simulink model "sm_car"  (R2025a)
settings: Solver=ode23t  StartTime=0.0  StopTime=400  MaxStep=0.4  RelTol=1e-3  AbsTol=1e-3  EnableMultiTasking=on
PreLoadFcn:
  | % Due to usability issue in Repeating Sequence block
  | warning('off','Simulink:Masking:Invalid');
  | 
  | % Eliminate unnecessary warnings in inactive variants
  | % Warnings generated only if you click through inactive variant
  | warning('off','MATLAB:nonExistentField');
  | warning('off','Simulink:Parameters:BlkParamUndefined');
PostLoadFcn:
  | set_param([bdroot '/Vehicle'],'popup_trailer','Off')
  | warning('off','sm:sli:setup:compile:LocalSolverNotSupported')
  | %sm_car_config_maneuver(bdroot,'WOT Braking');
  | sm_car_config_vehicle(bdroot,'false');
  | sm_car_config_logging(bdroot);
InitFcn:
  | sm_car_config_camera;
  | Vehicle = sm_car_vehcfg_checkConfig(Vehicle);
  | sm_car_check_tire_model(bdroot);
StartFcn:
  | tic;
StopFcn:
  | Elapsed_Sim_Time = toc;
  | % disp(['Elapsed Sim Time = ' num2str(Elapsed_Sim_Time)]);
undefined symbols (not defined in the file): Axle1D, AxleIn, Camera, Control, Driver, Free, Init, Maneuver, Pedal, RaceFix, RaceSpin, Scene, ShaftL1, ShaftL2, ShaftR1, ShaftR2, Soft, Stiff, Visual, X, xy_data_car_side, Y, Z
libraries: sm_lib x1546, nesl_utility x528, fl_lib x480, SimscapeFluids_lib x61, sdl_lib x49, simulink x29, ee_lib x7, simulink_extras x6, Linkage_Systems x4, Tire_1x2x x4, AntiRollBar_Systems x2, Linkage_Decoupled x2
(part 7 of 79)

== system sm_car/Driver/Closed Loop/Maneuver/PoseTarget Visual ==
  note: Allow yaw angle to wrap for
      | clockwise and counterclockwise laps.
  ref_z : Inport
  ref_y : Inport  Port=2
  ref_x : Inport  Port=3
  Lap Count : Inport  Port=4
  ref_ayaw : Inport  Port=5
  CW or CCW : Constant  Value=sign(Maneuver.Trajectory.aYaw.Value(end)-Maneuver.Trajectory.aYaw.Value(1))
  Gain : Gain  Gain=2*pi
  MechanismConfiguration : sm_lib/Utilities/Mechanism Configuration  UniformGravity=None  GravityVector=[0 0 -9.80665]  GravityVectorUnits=m/s^2  LinearizationDelta=0.001  JointModeTransitionNonlinearIterations=2
  Pace Car : Subsystem  mask(Car Body Geometry){whl_cutout_rad=0.5, whl_base=abs(Vehicle.Chassis.Body.sAxle1.Value(1)-Vehicle.Chassis.Body.sAxle2.Value(1)), thk_top=0.05, thk_side=0.05, car_track=Vehicle.Chassis.Body.Width.Value, offset_ref=[0 0 0.3225], extr_data_emblem_f=Visual.PaceCar.emblem.data*0.2, extr_data_emblem_r=Visual.PaceCar.emblem.data*0.2, clr_body_geo_top=Visual.PaceCar.body.clr, opc_body_geo_top=Visual.PaceCar.body.opc, clr_body_geo_left=Visual.PaceCar.body.clr, opc_body_geo_left=Visual.PaceCar.body.opc, clr_body_geo_right=Visual.PaceCar.body.clr, opc_body_geo_right=Visual.PaceCar.body.opc, clr_emblem_f=Visual.PaceCar.body.clr, opc_emblem_f=Visual.PaceCar.emblem.opc, clr_emblem_r=Visual.PaceCar.body.clr, opc_emblem_r=Visual.PaceCar.emblem.opc}
      mask prompts: whl_cutout_rad "Wheel Cutout Radius (m)"; whl_base "Wheelbase (m)"; thk_top "Top Thickness (m)"; thk_side "Side Thickness (m)"; car_track "Width (m)"; offset_ref "Offset to reference frame [xyz] (m)"; extr_data_emblem_f "Emblem Data Front [xy] (m)"; extr_data_emblem_r "Emblem Data Rear [xy] (m)"
      mask help: Creates simple car geometry. Adjusting the wheel cutout radius and wheelbase causes the profile to be adjusted. Press the Plot Profile button to see how the parameters affect the profile.
      mask init:
      | [xy_data_car_top xy_data_car_side] = Extr_Data_Car_Profile(whl_cutout_rad, whl_base,thk_top);
      mask TypeOptions extr_data_emblem_f:
      | Ornament
      | Front/ExtrusionCrossSection
      mask TypeOptions extr_data_emblem_r:
      | Ornament
      | Rear/ExtrusionCrossSection
      mask TypeOptions clr_body_geo_top: Top Surface/GraphicDiffuseColor
      mask TypeOptions opc_body_geo_top: Top Surface/GraphicOpacity
      mask TypeOptions clr_body_geo_left: Left Face/GraphicDiffuseColor
      mask TypeOptions opc_body_geo_left: Left Face/GraphicOpacity
      mask TypeOptions clr_body_geo_right: Right Face/GraphicDiffuseColor
      mask TypeOptions opc_body_geo_right: Right Face/GraphicOpacity
      mask TypeOptions clr_emblem_f:
      | Ornament
      | Front/GraphicDiffuseColor
      mask TypeOptions opc_emblem_f:
      | Ornament
      | Front/GraphicOpacity
      mask TypeOptions clr_emblem_r:
      | Ornament
      | Rear/GraphicDiffuseColor
      mask TypeOptions opc_emblem_r:
      | Ornament
      | Rear/GraphicOpacity
      mask DialogControl cont_geometry Prompt: Body Geometry
      mask DialogControl push_plot_profile Prompt: Plot Profile
      mask DialogControl push_plot_profile Callback:
      | v = get_param(gcb,'MaskWSVariables');
      | getMaskValue = containers.Map({v.Name}',{v.Value}');
      | evalin('base',...
      |     sprintf('Extr_Data_Car_Profile(%s,%s,%s,''%s'');',...
      |     num2str(getMaskValue('whl_cutout_rad')),...
      |     num2str(getMaskValue('whl_base')),...
      |     num2str(getMaskValue('thk_top')),'plot'));
      mask DialogControl cont_emblem Prompt: Emblem
      mask DialogControl cont_vis Prompt: Visualization
      mask DialogControl text_vis_clr Prompt: Color [RGB]
      mask DialogControl text_vis_opc Prompt: Opac. (0-1)
      mask DialogControl text_vis_top Prompt: Top
      mask DialogControl text_vis_left Prompt: Left Side
      mask DialogControl text_vis_right Prompt: Right Side
      mask DialogControl text_vis_emblem_f Prompt: Emblem Front
      mask DialogControl text_vis_emblem_r Prompt: Emblem Rear
      mask Display: image('sm_car_bodygeometry_sedan.png');
  Planar Joint : sm_lib/Joints/Planar Joint  JointMode=Normal  CompositeWrenchDir=FollowerOnBase  CompositeWrenchFrame=BaseFrame  SenseConstraintForce=off  SenseConstraintTorque=off  SenseTotalForce=off  SenseTotalTorque=off  PxPositionTargetSpecify=off  PxPositionTargetPriority=High  PxPositionTargetValue=0  PxPositionTargetValueUnits=m  PxVelocityTargetSpecify=off  PxVelocityTargetPriority=High  PxVelocityTargetValue=0  PxVelocityTargetValueUnits=m/s  PxEquilibriumPosition=0  PxEquilibriumPositionUnits=m  PxSpringStiffness=1  PxSpringStiffnessUnits=N/m  PxDampingCoefficient=1  PxDampingCoefficientUnits=N/(m/s)  PxLowerLimitSpecify=off  PxLowerLimitBound=-1  PxLowerLimitBoundUnits=m  PxLowerLimitStiffness=1e6  PxLowerLimitStiffnessUnits=N/m  PxLowerLimitDamping=1e3  PxLowerLimitDampingUnits=N/(m/s)  PxLowerLimitTransitionRegionWidth=1e-4  PxLowerLimitTransitionRegionWidthUnits=m  PxUpperLimitSpecify=off  PxUpperLimitBound=1  PxUpperLimitBoundUnits=m  PxUpperLimitStiffness=1e6  PxUpperLimitStiffnessUnits=N/m  PxUpperLimitDamping=1e3  PxUpperLimitDampingUnits=N/(m/s)  PxUpperLimitTransitionRegionWidth=1e-4  PxUpperLimitTransitionRegionWidthUnits=m  PxTorqueActuationMode=ComputedTorque  PxMotionActuationMode=InputMotion  PxSensePosition=off  PxSenseVelocity=off  PxSenseAcceleration=off  PxSenseTorqueForce=off  PxSenseLowerLimitTorqueForce=off  PxSenseUpperLimitTorqueForce=off  PyPositionTargetSpecify=off  PyPositionTargetPriority=High  PyPositionTargetValue=0  PyPositionTargetValueUnits=m  PyVelocityTargetSpecify=off  PyVelocityTargetPriority=High  PyVelocityTargetValue=0  PyVelocityTargetValueUnits=m/s  PyEquilibriumPosition=0  PyEquilibriumPositionUnits=m  PySpringStiffness=1  PySpringStiffnessUnits=N/m  PyDampingCoefficient=1  PyDampingCoefficientUnits=N/(m/s)  PyLowerLimitSpecify=off  PyLowerLimitBound=-1  PyLowerLimitBoundUnits=m  PyLowerLimitStiffness=1e6  PyLowerLimitStiffnessUnits=N/m  PyLowerLimitDamping=1e3  PyLowerLimitDampingUnits=N/(m/s)  PyLowerLimitTransitionRegionWidth=1e-4  PyLowerLimitTransitionRegionWidthUnits=m  PyUpperLimitSpecify=off  PyUpperLimitBound=1  PyUpperLimitBoundUnits=m  PyUpperLimitStiffness=1e6  PyUpperLimitStiffnessUnits=N/m  PyUpperLimitDamping=1e3  PyUpperLimitDampingUnits=N/(m/s)  PyUpperLimitTransitionRegionWidth=1e-4  PyUpperLimitTransitionRegionWidthUnits=m  PyTorqueActuationMode=ComputedTorque  PyMotionActuationMode=InputMotion  PySensePosition=off  PySenseVelocity=off  PySenseAcceleration=off  PySenseTorqueForce=off  PySenseLowerLimitTorqueForce=off  PySenseUpperLimitTorqueForce=off  RzPositionTargetSpecify=off  RzPositionTargetPriority=High  RzPositionTargetValue=0  RzPositionTargetValueUnits=deg  RzVelocityTargetSpecify=off  RzVelocityTargetPriority=High  RzVelocityTargetValue=0  RzVelocityTargetValueUnits=deg/s  RzEquilibriumPosition=0  RzEquilibriumPositionUnits=deg  RzSpringStiffness=1  RzSpringStiffnessUnits=N*m/deg  RzDampingCoefficient=1  RzDampingCoefficientUnits=N*m/(deg/s)  RzLowerLimitSpecify=off  RzLowerLimitBound=-90  RzLowerLimitBoundUnits=deg  RzLowerLimitStiffness=1e4  RzLowerLimitStiffnessUnits=N*m/deg  RzLowerLimitDamping=10  RzLowerLimitDampingUnits=N*m/(deg/s)  RzLowerLimitTransitionRegionWidth=0.1  RzLowerLimitTransitionRegionWidthUnits=deg  RzUpperLimitSpecify=off  RzUpperLimitBound=90  RzUpperLimitBoundUnits=deg  RzUpperLimitStiffness=1e4  RzUpperLimitStiffnessUnits=N*m/deg  RzUpperLimitDamping=10  RzUpperLimitDampingUnits=N*m/(deg/s)  RzUpperLimitTransitionRegionWidth=0.1  RzUpperLimitTransitionRegionWidthUnits=deg  RzTorqueActuationMode=ComputedTorque  RzMotionActuationMode=InputMotion  RzSensePosition=off  RzSenseVelocity=off  RzSenseAcceleration=off  RzSenseTorqueForce=off  RzSenseLowerLimitTorqueForce=off  RzSenseUpperLimitTorqueForce=off
  Prismatic Joint : sm_lib/Joints/Prismatic Joint  JointMode=Normal  CompositeWrenchDir=FollowerOnBase  CompositeWrenchFrame=BaseFrame  SenseConstraintForce=off  SenseConstraintTorque=off  SenseTotalForce=off  SenseTotalTorque=off  PositionTargetSpecify=off  PositionTargetPriority=High  PositionTargetValue=0  PositionTargetValueUnits=m  VelocityTargetSpecify=off  VelocityTargetPriority=High  VelocityTargetValue=0  VelocityTargetValueUnits=m/s  EquilibriumPosition=0  EquilibriumPositionUnits=m  SpringStiffness=0  SpringStiffnessUnits=N/m  DampingCoefficient=0  DampingCoefficientUnits=N/(m/s)  LowerLimitSpecify=off  LowerLimitBound=-1  LowerLimitBoundUnits=m  LowerLimitStiffness=1e6  LowerLimitStiffnessUnits=N/m  LowerLimitDamping=1e3  LowerLimitDampingUnits=N/(m/s)  LowerLimitTransitionRegionWidth=1e-4  LowerLimitTransitionRegionWidthUnits=m  UpperLimitSpecify=off  UpperLimitBound=1  UpperLimitBoundUnits=m  UpperLimitStiffness=1e6  UpperLimitStiffnessUnits=N/m  UpperLimitDamping=1e3  UpperLimitDampingUnits=N/(m/s)  UpperLimitTransitionRegionWidth=1e-4  UpperLimitTransitionRegionWidthUnits=m  TorqueActuationMode=ComputedTorque  MotionActuationMode=InputMotion  SensePosition=off  SenseVelocity=off  SenseAcceleration=off  SenseTorqueForce=off  SenseLowerLimitTorqueForce=off  SenseUpperLimitTorqueForce=off
  Product : Product
  Rigid Transform : sm_lib/Frames and Transforms/Rigid Transform  RotationMethod=None  FollAlignAxisA=+X  BaseAlignAxisA=+Y  FollAlignAxisB=+Y  BaseAlignAxisB=+Z  RotationStandardAxis=+Z  RotationAngle=0.0  RotationAngleUnits=deg  RotationArbitraryAxis=[0 0 1]  RotationSequenceAxes=FollowerAxes  RotationSequence=XYX  RotationSequenceAngles=[0 0 0]  RotationSequenceAnglesUnits=deg  RotationMatrix=[1 0 0; 0 1 0; 0 0 1]  Quaternion=[1 0 0 0]  TranslationMethod=Cartesian  TranslationCartesianOffset=[0 0 0.1]  TranslationCartesianOffsetUnits=m  TranslationStandardAxis=+Z  TranslationStandardOffset=0  TranslationStandardOffsetUnits=m  TranslationROffset=0  TranslationROffsetUnits=m  TranslationThetaOffset=0  TranslationThetaOffsetUnits=deg  TranslationZOffset=0  TranslationZOffsetUnits=m
  Simulink-PS Converter : nesl_utility/Simulink-PS Converter  PhysicalDomain=network_engine_domain  SubClassName=ps_input  LeftPortType=input  RightPortType=output  PseudoPeriodic=off  Frequencies=[]  NoiseDistribution=none  NoiseParameters=[]  Unit=1  AffineConversion=off  FilteringAndDerivatives=filter  SimscapeFilterOrder=2  InputFilterTimeConstant=0.1  UdotUserProvided=0
  Simulink-PS Converter1 : nesl_utility/Simulink-PS Converter  PhysicalDomain=network_engine_domain  SubClassName=ps_input  LeftPortType=input  RightPortType=output  PseudoPeriodic=off  Frequencies=[]  NoiseDistribution=none  NoiseParameters=[]  Unit=1  AffineConversion=off  FilteringAndDerivatives=filter  SimscapeFilterOrder=2  InputFilterTimeConstant=0.1  UdotUserProvided=0
  Simulink-PS Converter2 : nesl_utility/Simulink-PS Converter  PhysicalDomain=network_engine_domain  SubClassName=ps_input  LeftPortType=input  RightPortType=output  PseudoPeriodic=off  Frequencies=[]  NoiseDistribution=none  NoiseParameters=[]  Unit=rad  AffineConversion=off  FilteringAndDerivatives=filter  SimscapeFilterOrder=2  InputFilterTimeConstant=0.1  UdotUserProvided=0
  Simulink-PS Converter3 : nesl_utility/Simulink-PS Converter  PhysicalDomain=network_engine_domain  SubClassName=ps_input  LeftPortType=input  RightPortType=output  PseudoPeriodic=off  Frequencies=[]  NoiseDistribution=none  NoiseParameters=[]  Unit=1  AffineConversion=off  FilteringAndDerivatives=filter  SimscapeFilterOrder=2  InputFilterTimeConstant=0.1  UdotUserProvided=0
  Solver Configuration : nesl_utility/Solver Configuration  PhysicalDomain=network_engine_domain  SubClassName=solver  LeftPortType=input  RightPortType=generic  Tones=[]  Harmonics=[]  SimulateNoise=off  Profile=off  UseLocalSampling=off  EnableSwitchedLinearOptims=on  FrequencyDomain=off  UseCCode=off  RelTol=0.001  AbsTol=1e-06  MinStep=1e-09  ToWorkspace=off  RevertToSquareIcSolve=off  NumHomotopyIterations=100  PhasorMode=off  PhasorModeNumHarmonics=1  ConsistencySolver=NEWTON_FTOL  IndexReductionMethod=DerivativeReplacement  DoDC=off  ResidualTolerance=1e-9  ConsistencyTolSource=GLOBAL  ConsistencyAbsTol=0.001  ConsistencyRelTol=0.001  ConsistencyTolFactor=0.001  UseLocalSolver=off  LocalSolverChoice=NE_BACKWARD_EULER_ADVANCER  ResolveIndetEquations=on  FunctionEvalNumThread=1  LocalSolverSampleTime=0.001  DoFixedCost=off  MaxNonlinIter=5  MaxModeIter=2  ComputeImpulses=off  ImpulseIterations=2  LinearAlgebra=Sparse  LinearAlgebraNumThread=0  EquationFormulation=NE_TIME_EF  DelaysMemoryBudget=1024  AutomaticFiltering=on  FilteringTimeConstant=0.001  PartitionStorageMethod=AS_NEEDED  PartitionMemoryBudget=1024  PartitionMethod=FAST  MultibodyUseLocalSolver=off  MultibodyLocalSolverChoice=ODE1  MultibodyLocalSolverSampleTime=0.001
  Sum : Sum  Inputs=|++
  World Frame : sm_lib/Frames and Transforms/World Frame
  wires:
  CW or CCW/1 -> Product/2
  Gain/1 -> Product/1
  Sum/1 -> Simulink-PS Converter2/1
  Product/1 -> Sum/2
  Lap Count/1 -> Gain/1
  ref_ayaw/1 -> Sum/1
  ref_y/1 -> Simulink-PS Converter1/1
  ref_x/1 -> Simulink-PS Converter/1
  ref_z/1 -> Simulink-PS Converter3/1
  connections:
  Pace Car/LConn1 -- Rigid Transform/RConn1
  Simulink-PS Converter/RConn1 -- Planar Joint/LConn2
  Simulink-PS Converter2/RConn1 -- Planar Joint/LConn4
  Rigid Transform/LConn1 -- Prismatic Joint/RConn1
  Simulink-PS Converter1/RConn1 -- Planar Joint/LConn3
  World Frame/RConn1 -- Planar Joint/LConn1 -- MechanismConfiguration/RConn1 -- Solver Configuration/RConn1
  Prismatic Joint/LConn1 -- Planar Joint/RConn1
  Simulink-PS Converter3/RConn1 -- Prismatic Joint/LConn2

== system sm_car/Driver/Closed Loop/Maneuver/vx override ==
  note: Override speed signal using
      | gain (to set to zero) and/or with an
      | offset (for passing maneuver).
  vx : Inport
  Bus Selector2 : BusSelector  OutputSignals=offset,gain
  Constant5 : Constant  Value=Maneuver.Trajectory.vx.Value
  Product : Product
  Sum : Sum  Inputs=++|
  vx_ovr : Outport  VectorParamsAs1DForOutWhenUnconnected=off
  wires:
  Bus Selector2/1 -> Sum/1  "<offset>"
  Product/1 -> Sum/2
  Constant5/1 -> Product/2
  Sum/1 -> vx_ovr/1
  Bus Selector2/2 -> Product/1  "<gain>"
  vx/1 -> Bus Selector2/1

== system sm_car/Driver/Closed Loop/Maneuver/x override ==
  note: Override speed signal using
      | gain (to set to zero) and/or with an
      | offset (for passing maneuver).
  x : Inport
  Bus Selector2 : BusSelector  OutputSignals=offset,gain
  Constant3 : Constant  Value=Maneuver.Trajectory.x.Value
  Product : Product
  Sum : Sum  Inputs=++|
  x_ovr : Outport  VectorParamsAs1DForOutWhenUnconnected=off
  wires:
  x/1 -> Bus Selector2/1
  Bus Selector2/2 -> Product/1  "<gain>"
  Sum/1 -> x_ovr/1
  Constant3/1 -> Product/2
  Product/1 -> Sum/2
  Bus Selector2/1 -> Sum/1  "<offset>"

== system sm_car/Driver/Closed Loop/Maneuver/y override ==
  note: Override speed signal using
      | gain (to set to zero) and/or with an
      | offset (for passing maneuver).
  y : Inport
  Bus Selector2 : BusSelector  OutputSignals=offset,gain
  Constant4 : Constant  Value=Maneuver.Trajectory.y.Value
  Product : Product
  Sum : Sum  Inputs=++|
  y_ovr : Outport  VectorParamsAs1DForOutWhenUnconnected=off
  wires:
  Bus Selector2/1 -> Sum/1  "<offset>"
  Product/1 -> Sum/2
  Constant4/1 -> Product/2
  Sum/1 -> y_ovr/1
  Bus Selector2/2 -> Product/1  "<gain>"
  y/1 -> Bus Selector2/1

== system sm_car/Driver/Closed Loop/Maneuver/z override ==
  note: Override speed signal using
      | gain (to set to zero) and/or with an
      | offset (for passing maneuver).
  z : Inport
  Bus Selector2 : BusSelector  OutputSignals=offset,gain
  Constant1 : Constant  Value=Maneuver.Trajectory.z.Value
  Product : Product
  Sum : Sum  Inputs=++|
  z_ovr : Outport  VectorParamsAs1DForOutWhenUnconnected=off
  wires:
  z/1 -> Bus Selector2/1
  Bus Selector2/2 -> Product/1  "<gain>"
  Sum/1 -> z_ovr/1
  Constant1/1 -> Product/2
  Product/1 -> Sum/2
  Bus Selector2/1 -> Sum/1  "<offset>"

== system sm_car/Driver/Closed Loop/Override/None ==
  dist : Inport
  Obs : Inport  Port=2
  Bus Creator{,2..4} (4 alike) : BusCreator  Inputs=2
  Bus Creator1 : BusCreator  Inputs=4
  Constant{1..2,4,6} (4 alike) : Constant  Value=0
  Constant{3,5,7..8} (4 alike) : Constant
  Terminator : Terminator
  Terminator1 : Terminator
  Ovr : Outport  VectorParamsAs1DForOutWhenUnconnected=off
  wires:
  Bus Creator4/1 -> Bus Creator1/1  "x"
  Bus Creator/1 -> Bus Creator1/4  "vx"
  Bus Creator3/1 -> Bus Creator1/2  "y"
  Constant2/1 -> Bus Creator2/1  "offset"
  Bus Creator2/1 -> Bus Creator1/3  "z"
  Constant3/1 -> Bus Creator2/2  "gain"
  Constant4/1 -> Bus Creator3/1  "offset"
  Constant5/1 -> Bus Creator3/2  "gain"
  Constant7/1 -> Bus Creator4/2  "gain"
  Constant6/1 -> Bus Creator4/1  "offset"
  Constant8/1 -> Bus Creator/2  "gain"
  Constant1/1 -> Bus Creator/1  "offset"
  Bus Creator1/1 -> Ovr/1
  Obs/1 -> Terminator1/1
  dist/1 -> Terminator/1

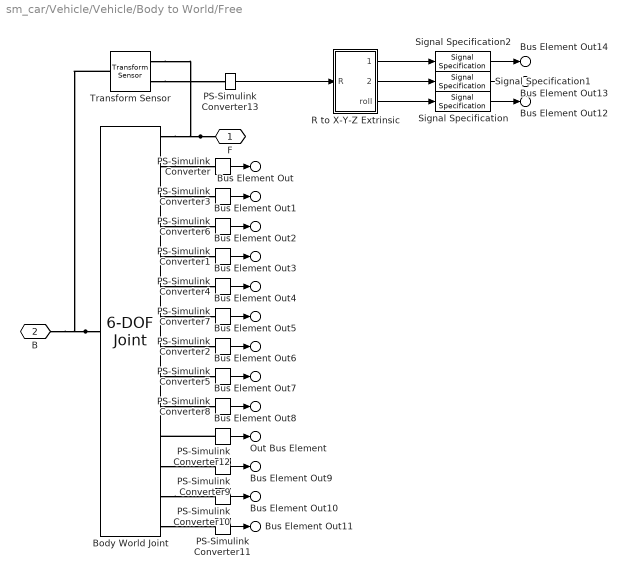
== system sm_car/Vehicle/Vehicle/Body to World/Free ==
  Body World Joint : sm_lib/Joints/6-DOF Joint  JointMode=Normal  CompositeWrenchDir=FollowerOnBase  CompositeWrenchFrame=BaseFrame  SenseConstraintForce=off  SenseConstraintTorque=off  SenseTotalForce=off  SenseTotalTorque=off  PxPositionTargetSpecify=on  PxPositionTargetPriority=Low  PxPositionTargetValue=Init.sChassis.Value(1)  PxPositionTargetValueUnits=m  PxVelocityTargetSpecify=on  PxVelocityTargetPriority=Low  PxVelocityTargetValue=initial_vveh(1)  PxVelocityTargetValueUnits=m/s  PxEquilibriumPosition=0  PxEquilibriumPositionUnits=m  PxSpringStiffness=0  PxSpringStiffnessUnits=N/m  PxDampingCoefficient=0  PxDampingCoefficientUnits=N/(m/s)  PxLowerLimitSpecify=off  PxLowerLimitBound=-1  PxLowerLimitBoundUnits=m  PxLowerLimitStiffness=1e6  PxLowerLimitStiffnessUnits=N/m  PxLowerLimitDamping=1e3  PxLowerLimitDampingUnits=N/(m/s)  PxLowerLimitTransitionRegionWidth=1e-4  PxLowerLimitTransitionRegionWidthUnits=m  PxUpperLimitSpecify=off  PxUpperLimitBound=1  PxUpperLimitBoundUnits=m  PxUpperLimitStiffness=1e6  PxUpperLimitStiffnessUnits=N/m  PxUpperLimitDamping=1e3  PxUpperLimitDampingUnits=N/(m/s)  PxUpperLimitTransitionRegionWidth=1e-4  PxUpperLimitTransitionRegionWidthUnits=m  PxTorqueActuationMode=NoTorque  PxMotionActuationMode=ComputedMotion  PxSensePosition=on  PxSenseVelocity=on  PxSenseAcceleration=on  PxSenseTorqueForce=off  PxSenseLowerLimitTorqueForce=off  PxSenseUpperLimitTorqueForce=off  PyPositionTargetSpecify=on  PyPositionTargetPriority=Low  PyPositionTargetValue=Init.sChassis.Value(2)  PyPositionTargetValueUnits=m  PyVelocityTargetSpecify=on  PyVelocityTargetPriority=Low  PyVelocityTargetValue=initial_vveh(2)  PyVelocityTargetValueUnits=m/s  PyEquilibriumPosition=0  PyEquilibriumPositionUnits=m  PySpringStiffness=0  PySpringStiffnessUnits=N/m  PyDampingCoefficient=0  PyDampingCoefficientUnits=N/(m/s)  PyLowerLimitSpecify=off  PyLowerLimitBound=-1  PyLowerLimitBoundUnits=m  PyLowerLimitStiffness=1e6  PyLowerLimitStiffnessUnits=N/m  PyLowerLimitDamping=1e3  PyLowerLimitDampingUnits=N/(m/s)  PyLowerLimitTransitionRegionWidth=1e-4  PyLowerLimitTransitionRegionWidthUnits=m  PyUpperLimitSpecify=off  PyUpperLimitBound=1  PyUpperLimitBoundUnits=m  PyUpperLimitStiffness=1e6  PyUpperLimitStiffnessUnits=N/m  PyUpperLimitDamping=1e3  PyUpperLimitDampingUnits=N/(m/s)  PyUpperLimitTransitionRegionWidth=1e-4  PyUpperLimitTransitionRegionWidthUnits=m  PyTorqueActuationMode=NoTorque  PyMotionActuationMode=ComputedMotion  PySensePosition=on  PySenseVelocity=on  PySenseAcceleration=on  PySenseTorqueForce=off  PySenseLowerLimitTorqueForce=off  PySenseUpperLimitTorqueForce=off  PzPositionTargetSpecify=on  PzPositionTargetPriority=Low  PzPositionTargetValue=Init.sChassis.Value(3)  PzPositionTargetValueUnits=m  PzVelocityTargetSpecify=on  PzVelocityTargetPriority=Low  PzVelocityTargetValue=initial_vveh(3)  PzVelocityTargetValueUnits=m/s  PzEquilibriumPosition=0  PzEquilibriumPositionUnits=m  PzSpringStiffness=0  PzSpringStiffnessUnits=N/m  PzDampingCoefficient=0  PzDampingCoefficientUnits=N/(m/s)  PzLowerLimitSpecify=off  PzLowerLimitBound=-1  PzLowerLimitBoundUnits=m  PzLowerLimitStiffness=1e6  PzLowerLimitStiffnessUnits=N/m  PzLowerLimitDamping=1e3  PzLowerLimitDampingUnits=N/(m/s)  PzLowerLimitTransitionRegionWidth=1e-4  PzLowerLimitTransitionRegionWidthUnits=m  PzUpperLimitSpecify=off  PzUpperLimitBound=1  PzUpperLimitBoundUnits=m  PzUpperLimitStiffness=1e6  PzUpperLimitStiffnessUnits=N/m  PzUpperLimitDamping=1e3  PzUpperLimitDampingUnits=N/(m/s)  PzUpperLimitTransitionRegionWidth=1e-4  PzUpperLimitTransitionRegionWidthUnits=m  PzTorqueActuationMode=NoTorque  PzMotionActuationMode=ComputedMotion  PzSensePosition=on  PzSenseVelocity=on  PzSenseAcceleration=on  PzSenseTorqueForce=off  PzSenseLowerLimitTorqueForce=off  PzSenseUpperLimitTorqueForce=off  SphPositionTargetSpecify=on  SphPositionTargetPriority=Low  SphPositionTargetRotationMethod=RotationSequence  SphPositionTargetFollAlignAxisA=+X  SphPositionTargetBaseAlignAxisA=+Y  SphPositionTargetFollAlignAxisB=+Y  SphPositionTargetBaseAlignAxisB=+Z  SphPositionTargetRotationStandardAxis=+Z  SphPositionTargetRotationAngle=0.0  SphPositionTargetRotationAngleUnits=deg  SphPositionTargetRotationArbitraryAxis=[0 0 1]  SphPositionTargetRotationSequenceAxes=FollowerAxes  SphPositionTargetRotationSequence=ZYX  SphPositionTargetRotationSequenceAngles=initial_aveh  SphPositionTargetRotationSequenceAnglesUnits=rad  SphPositionTargetRotationMatrix=[1 0 0; 0 1 0; 0 0 1]  SphPositionTargetQuaternion=[1 0 0 0]  SphVelocityTargetSpecify=on  SphVelocityTargetPriority=Low  SphVelocityTargetValue=[0 0 0]  SphVelocityTargetValueUnits=deg/s  SphVelocityTargetInFollowerFrame=on  SphEqPosRotationMethod=None  SphEqPosFollAlignAxisA=+X  SphEqPosBaseAlignAxisA=+Y  SphEqPosFollAlignAxisB=+Y  SphEqPosBaseAlignAxisB=+Z  SphEqPosRotationStandardAxis=+Z  SphEqPosRotationAngle=0.0  SphEqPosRotationAngleUnits=deg  SphEqPosRotationArbitraryAxis=[0 0 1]  SphEqPosRotationSequenceAxes=FollowerAxes  SphEqPosRotationSequence=XYX  SphEqPosRotationSequenceAngles=[0 0 0]  SphEqPosRotationSequenceAnglesUnits=deg  SphEqPosRotationMatrix=[1 0 0; 0 1 0; 0 0 1]  SphEqPosQuaternion=[1 0 0 0]  SphSpringStiffness=0  SphSpringStiffnessUnits=N*m/deg  SphDampingCoefficient=0  SphDampingCoefficientUnits=N*m/(deg/s)  SphLowerLimitSpecify=off  SphLowerLimitBound=15  SphLowerLimitBoundUnits=deg  SphLowerLimitStiffness=1e4  SphLowerLimitStiffnessUnits=N*m/deg  SphLowerLimitDamping=10  SphLowerLimitDampingUnits=N*m/(deg/s)  SphLowerLimitTransitionRegionWidth=0.1  SphLowerLimitTransitionRegionWidthUnits=deg  SphUpperLimitSpecify=off  SphUpperLimitBound=45  SphUpperLimitBoundUnits=deg  SphUpperLimitStiffness=1e4  SphUpperLimitStiffnessUnits=N*m/deg  SphUpperLimitDamping=10  SphUpperLimitDampingUnits=N*m/(deg/s)  SphUpperLimitTransitionRegionWidth=0.1  SphUpperLimitTransitionRegionWidthUnits=deg  SphTorqueActuationMode=NoTorque  SphActuateTorqueX=off  SphActuateTorqueY=off  SphActuateTorqueZ=off  SphActuateTorque=off  SphActuationFrame=BaseFrame  SphSensePosition=on  SphSenseVelocityX=on  SphSenseVelocityY=on  SphSenseVelocityZ=on  SphSenseVelocity=off  SphSenseAccelerationX=off  SphSenseAccelerationY=off  SphSenseAccelerationZ=off  SphSenseAcceleration=off  SphSenseLowerLimitTorqueMag=off  SphSenseUpperLimitTorqueMag=off  SphSensingFrame=BaseFrame
  PS-Simulink Converter : nesl_utility/PS-Simulink Converter  PhysicalDomain=network_engine_domain  SubClassName=ps_output  LeftPortType=input  RightPortType=output  PseudoPeriodic=off  Frequencies=[]  VectorFormat=1-D array  Unit=m  AffineConversion=off
  PS-Simulink Converter1 : nesl_utility/PS-Simulink Converter  PhysicalDomain=network_engine_domain  SubClassName=ps_output  LeftPortType=input  RightPortType=output  PseudoPeriodic=off  Frequencies=[]  VectorFormat=1-D array  Unit=m  AffineConversion=off
  PS-Simulink Converter10 : nesl_utility/PS-Simulink Converter  PhysicalDomain=network_engine_domain  SubClassName=ps_output  LeftPortType=input  RightPortType=output  PseudoPeriodic=off  Frequencies=[]  VectorFormat=1-D array  Unit=rad/s  AffineConversion=off
  PS-Simulink Converter11 : nesl_utility/PS-Simulink Converter  PhysicalDomain=network_engine_domain  SubClassName=ps_output  LeftPortType=input  RightPortType=output  PseudoPeriodic=off  Frequencies=[]  VectorFormat=1-D array  Unit=rad/s  AffineConversion=off
  PS-Simulink Converter12 : nesl_utility/PS-Simulink Converter  PhysicalDomain=network_engine_domain  SubClassName=ps_output  LeftPortType=input  RightPortType=output  PseudoPeriodic=off  Frequencies=[]  VectorFormat=1-D array  Unit=1  AffineConversion=off
  PS-Simulink Converter13 : nesl_utility/PS-Simulink Converter  PhysicalDomain=network_engine_domain  SubClassName=ps_output  LeftPortType=input  RightPortType=output  PseudoPeriodic=off  Frequencies=[]  VectorFormat=1-D array  Unit=1  AffineConversion=off
  PS-Simulink Converter2 : nesl_utility/PS-Simulink Converter  PhysicalDomain=network_engine_domain  SubClassName=ps_output  LeftPortType=input  RightPortType=output  PseudoPeriodic=off  Frequencies=[]  VectorFormat=1-D array  Unit=m  AffineConversion=off
  PS-Simulink Converter3 : nesl_utility/PS-Simulink Converter  PhysicalDomain=network_engine_domain  SubClassName=ps_output  LeftPortType=input  RightPortType=output  PseudoPeriodic=off  Frequencies=[]  VectorFormat=1-D array  Unit=m/s  AffineConversion=off
  PS-Simulink Converter4 : nesl_utility/PS-Simulink Converter  PhysicalDomain=network_engine_domain  SubClassName=ps_output  LeftPortType=input  RightPortType=output  PseudoPeriodic=off  Frequencies=[]  VectorFormat=1-D array  Unit=m/s  AffineConversion=off
  PS-Simulink Converter5 : nesl_utility/PS-Simulink Converter  PhysicalDomain=network_engine_domain  SubClassName=ps_output  LeftPortType=input  RightPortType=output  PseudoPeriodic=off  Frequencies=[]  VectorFormat=1-D array  Unit=m/s  AffineConversion=off
  PS-Simulink Converter6 : nesl_utility/PS-Simulink Converter  PhysicalDomain=network_engine_domain  SubClassName=ps_output  LeftPortType=input  RightPortType=output  PseudoPeriodic=off  Frequencies=[]  VectorFormat=1-D array  Unit=m/s^2  AffineConversion=off
  PS-Simulink Converter7 : nesl_utility/PS-Simulink Converter  PhysicalDomain=network_engine_domain  SubClassName=ps_output  LeftPortType=input  RightPortType=output  PseudoPeriodic=off  Frequencies=[]  VectorFormat=1-D array  Unit=m/s^2  AffineConversion=off
  PS-Simulink Converter8 : nesl_utility/PS-Simulink Converter  PhysicalDomain=network_engine_domain  SubClassName=ps_output  LeftPortType=input  RightPortType=output  PseudoPeriodic=off  Frequencies=[]  VectorFormat=1-D array  Unit=m/s^2  AffineConversion=off
  PS-Simulink Converter9 : nesl_utility/PS-Simulink Converter  PhysicalDomain=network_engine_domain  SubClassName=ps_output  LeftPortType=input  RightPortType=output  PseudoPeriodic=off  Frequencies=[]  VectorFormat=1-D array  Unit=rad/s  AffineConversion=off
  R to X-Y-Z Extrinsic : Subsystem  mask(Rotation Matrix to X-Y-Z Extrinsic){}
      mask help: Computes roll / pitch / yaw values assuming they correspond to X, Y, and Z rotations, applied in that order and using extrinsic rotations (rotations applied about the fixed axes of the base frame). Does not handle case where Y (pitch) rotation is +/-90 degrees.
  Signal Specification : SignalSpecification  Unit=rad
  Signal Specification1 : SignalSpecification  Unit=rad
  Signal Specification2 : SignalSpecification  Unit=rad
  Transform Sensor : sm_lib/Frames and Transforms/Transform Sensor  MeasurementFrame=World  RotationSequence=XYX  SenseAngle=off  SenseAxis=off  SenseQ=off  SenseR=on  SenseRotationSequence=off  SenseOmegaX=off  SenseOmegaY=off  SenseOmegaZ=off  SenseOmega=off  SenseQDot=off  SenseRDot=off  SenseRotationSequenceDot=off  SenseAlphaX=off  SenseAlphaY=off  SenseAlphaZ=off  SenseAlpha=off  SenseQDDot=off  SenseRDDot=off  SenseX=off  SenseY=off  SenseZ=off  SenseXYZ=off  SenseRad=off  SenseAzim=off  SenseDist=off  SenseInc=off  SenseXDot=off  SenseYDot=off  SenseZDot=off  SenseXYZDot=off  SenseRadDot=off  SenseAzimDot=off  SenseDistDot=off  SenseIncDot=off  SenseXDDot=off  SenseYDDot=off  SenseZDDot=off  SenseXYZDDot=off  SenseRadDDot=off  SenseAzimDDot=off  SenseDistDDot=off  SenseIncDDot=off
  F : PMIOPort  Side=Left
  B : PMIOPort  Port=2  Side=Right
  Bus Element Out : Outport  VectorParamsAs1DForOutWhenUnconnected=off  PortName=World  Element=x
  Bus Element Out3 : Outport  VectorParamsAs1DForOutWhenUnconnected=off  PortName=World  Element=y
  Bus Element Out6 : Outport  VectorParamsAs1DForOutWhenUnconnected=off  PortName=World  Element=z
  Bus Element Out1 : Outport  VectorParamsAs1DForOutWhenUnconnected=off  PortName=World  Element=vx
  Bus Element Out4 : Outport  VectorParamsAs1DForOutWhenUnconnected=off  PortName=World  Element=vy
  Bus Element Out7 : Outport  VectorParamsAs1DForOutWhenUnconnected=off  PortName=World  Element=vz
  Bus Element Out2 : Outport  VectorParamsAs1DForOutWhenUnconnected=off  PortName=World  Element=gx
  Bus Element Out5 : Outport  VectorParamsAs1DForOutWhenUnconnected=off  PortName=World  Element=gy
  Bus Element Out8 : Outport  VectorParamsAs1DForOutWhenUnconnected=off  PortName=World  Element=gz
  Bus Element Out9 : Outport  VectorParamsAs1DForOutWhenUnconnected=off  PortName=World  Element=nRoll
  Bus Element Out10 : Outport  VectorParamsAs1DForOutWhenUnconnected=off  PortName=World  Element=nPitch
  Bus Element Out11 : Outport  VectorParamsAs1DForOutWhenUnconnected=off  PortName=World  Element=nYaw
  Bus Element Out12 : Outport  VectorParamsAs1DForOutWhenUnconnected=off  PortName=World  Element=aRoll
  Bus Element Out13 : Outport  VectorParamsAs1DForOutWhenUnconnected=off  PortName=World  Element=aPitch
  Bus Element Out14 : Outport  VectorParamsAs1DForOutWhenUnconnected=off  PortName=World  Element=aYaw
  Out Bus Element : Outport  VectorParamsAs1DForOutWhenUnconnected=off  PortName=World  Element=Q
  wires:
  R to X-Y-Z Extrinsic/1(yaw) -> Signal Specification2/1
  R to X-Y-Z Extrinsic/3(roll) -> Signal Specification/1
  R to X-Y-Z Extrinsic/2(pitch) -> Signal Specification1/1
  PS-Simulink Converter13/1 -> R to X-Y-Z Extrinsic/1(R)
  PS-Simulink Converter12/1 -> Out Bus Element/1
  PS-Simulink Converter11/1 -> Bus Element Out11/1
  PS-Simulink Converter10/1 -> Bus Element Out10/1
  Signal Specification/1 -> Bus Element Out12/1
  Signal Specification1/1 -> Bus Element Out13/1
  Signal Specification2/1 -> Bus Element Out14/1
  PS-Simulink Converter3/1 -> Bus Element Out1/1
  PS-Simulink Converter2/1 -> Bus Element Out6/1
  PS-Simulink Converter6/1 -> Bus Element Out2/1
  PS-Simulink Converter4/1 -> Bus Element Out4/1
  PS-Simulink Converter/1 -> Bus Element Out/1
  PS-Simulink Converter5/1 -> Bus Element Out7/1
  PS-Simulink Converter9/1 -> Bus Element Out9/1
  PS-Simulink Converter8/1 -> Bus Element Out8/1
  PS-Simulink Converter7/1 -> Bus Element Out5/1
  PS-Simulink Converter1/1 -> Bus Element Out3/1
  connections:
  Transform Sensor/RConn2 -- PS-Simulink Converter13/LConn1
  PS-Simulink Converter12/LConn1 -- Body World Joint/RConn11
  Body World Joint/RConn8 -- PS-Simulink Converter2/LConn1
  Body World Joint/RConn9 -- PS-Simulink Converter5/LConn1
  F/RConn1 -- Transform Sensor/RConn1 -- Body World Joint/RConn1
  Body World Joint/RConn3 -- PS-Simulink Converter3/LConn1
  Body World Joint/RConn10 -- PS-Simulink Converter8/LConn1
  Body World Joint/RConn4 -- PS-Simulink Converter6/LConn1
  Body World Joint/RConn2 -- PS-Simulink Converter/LConn1
  Body World Joint/RConn7 -- PS-Simulink Converter7/LConn1
  Body World Joint/RConn13 -- PS-Simulink Converter10/LConn1
  Body World Joint/RConn14 -- PS-Simulink Converter11/LConn1
  Body World Joint/RConn5 -- PS-Simulink Converter1/LConn1
  Body World Joint/LConn1 -- Transform Sensor/LConn1 -- B/RConn1
  Body World Joint/RConn12 -- PS-Simulink Converter9/LConn1
  Body World Joint/RConn6 -- PS-Simulink Converter4/LConn1

== system sm_car/Vehicle/Vehicle/Brakes/PedalAbstract DiscDisc ==
  In Bus Element5 : Inport  PortName=DrvBus  Element=rBrakePedal
  In Bus Element1 : Inport  Port=2  PortName=CtrlBus
  Actuator L1 : Subsystem  mask(Brake Actuator, Pedal Input){brk_max_p=brk_max_p_a1, brk_filt=brk_filt_a1}
      mask prompts: brk_max_p "Max Pad Pressure (Pa)"; brk_filt "Time Constant (s)"
      mask help: Models brake actuator dynamics. A transfer function models delay from brake pedal movement to pressure applied at brake rotor.
      mask TypeOptions brk_max_p: Filter/Numerator
  Actuator L2 : Subsystem  mask(Brake Actuator, Pedal Input){brk_max_p=brk_max_p_a2, brk_filt=brk_filt_a2}
      mask prompts: brk_max_p "Max Pad Pressure (Pa)"; brk_filt "Time Constant (s)"
      mask help: Models brake actuator dynamics. A transfer function models delay from brake pedal movement to pressure applied at brake rotor.
      mask TypeOptions brk_max_p: Filter/Numerator
  Actuator R1 : Subsystem  mask(Brake Actuator, Pedal Input){brk_max_p=brk_max_p_a1, brk_filt=brk_filt_a1}
      mask prompts: brk_max_p "Max Pad Pressure (Pa)"; brk_filt "Time Constant (s)"
      mask help: Models brake actuator dynamics. A transfer function models delay from brake pedal movement to pressure applied at brake rotor.
      mask TypeOptions brk_max_p: Filter/Numerator
  Actuator R2 : Subsystem  mask(Brake Actuator, Pedal Input){brk_max_p=brk_max_p_a2, brk_filt=brk_filt_a2}
      mask prompts: brk_max_p "Max Pad Pressure (Pa)"; brk_filt "Time Constant (s)"
      mask help: Models brake actuator dynamics. A transfer function models delay from brake pedal movement to pressure applied at brake rotor.
      mask TypeOptions brk_max_p: Filter/Numerator
  Disc Brake L1 : sdl_lib/Brakes & Detents/Rotational/Disc Brake  r_mean=brk_pad_rad_a1 m  bore=brk_cyl_bore_a1 m  n_pads=brk_n_pads_a1  thermal_port=simscape.enum.thermaleffects.omit  mu_static=brk_mu_static_a1  mu_coulomb=brk_mu_kin_a1  temperature_TLU=[280, 300, 320] K  mu_static_TLU=[.9, .8, .7]  mu_coulomb_TLU=[.8, .7, .6]  brkwy_vel=brk_trans_vel_a1 rad/s  visc_coef=brk_visc_coef_a1 N*m/(rad/s)  thermal_mass=50 kJ/K  temperature_specify=off  temperature_priority=High  temperature=300 K  temperature_nominal_specify=off  temperature_nominal_value=1  temperature_nominal_unit=K
  Disc Brake L2 : sdl_lib/Brakes & Detents/Rotational/Disc Brake  r_mean=brk_pad_rad_a2 m  bore=brk_cyl_bore_a2 m  n_pads=brk_n_pads_a2  thermal_port=simscape.enum.thermaleffects.omit  mu_static=brk_mu_static_a2  mu_coulomb=brk_mu_kin_a2  temperature_TLU=[280, 300, 320] K  mu_static_TLU=[.9, .8, .7]  mu_coulomb_TLU=[.8, .7, .6]  brkwy_vel=brk_trans_vel_a2 rad/s  visc_coef=brk_visc_coef_a2 N*m/(rad/s)  thermal_mass=50 kJ/K  temperature_specify=off  temperature_priority=High  temperature=300 K  temperature_nominal_specify=off  temperature_nominal_value=1  temperature_nominal_unit=K
  Disc Brake R1 : sdl_lib/Brakes & Detents/Rotational/Disc Brake  r_mean=brk_pad_rad_a1 m  bore=brk_cyl_bore_a1 m  n_pads=brk_n_pads_a1  thermal_port=simscape.enum.thermaleffects.omit  mu_static=brk_mu_static_a1  mu_coulomb=brk_mu_kin_a1  temperature_TLU=[280, 300, 320] K  mu_static_TLU=[.9, .8, .7]  mu_coulomb_TLU=[.8, .7, .6]  brkwy_vel=brk_trans_vel_a1 rad/s  visc_coef=brk_visc_coef_a1 N*m/(rad/s)  thermal_mass=50 kJ/K  temperature_specify=off  temperature_priority=High  temperature=300 K  temperature_nominal_specify=off  temperature_nominal_value=1  temperature_nominal_unit=K
  Disc Brake R2 : sdl_lib/Brakes & Detents/Rotational/Disc Brake  r_mean=brk_pad_rad_a2 m  bore=brk_cyl_bore_a2 m  n_pads=brk_n_pads_a2  thermal_port=simscape.enum.thermaleffects.omit  mu_static=brk_mu_static_a2  mu_coulomb=brk_mu_kin_a2  temperature_TLU=[280, 300, 320] K  mu_static_TLU=[.9, .8, .7]  mu_coulomb_TLU=[.8, .7, .6]  brkwy_vel=brk_trans_vel_a2 rad/s  visc_coef=brk_visc_coef_a2 N*m/(rad/s)  thermal_mass=50 kJ/K  temperature_specify=off  temperature_priority=High  temperature=300 K  temperature_nominal_specify=off  temperature_nominal_value=1  temperature_nominal_unit=K
  Sensing Torque L1 : Subsystem
  Sensing Torque L2 : Subsystem
  Sensing Torque R1 : Subsystem
  Sensing Torque R2 : Subsystem
  Simscape Bus L1 : SimscapeBus  HierarchyStrings=Axle1D
  Simscape Bus L2 : SimscapeBus  HierarchyStrings=Axle1D
  Simscape Bus R1 : SimscapeBus  HierarchyStrings=Axle1D
  Simscape Bus R2 : SimscapeBus  HierarchyStrings=Axle1D
  Terminator : Terminator
  L1 : PMIOPort  Side=Left
  R1 : PMIOPort  Port=2  Side=Right
  L2 : PMIOPort  Port=3  Side=Left
  R2 : PMIOPort  Port=4  Side=Right
  Out Bus Element2 : Outport  VectorParamsAs1DForOutWhenUnconnected=off  PortName=OutB  Element=MBrakeL1
  Out Bus Element : Outport  VectorParamsAs1DForOutWhenUnconnected=off  PortName=OutB  Element=MBrakeR1
  Out Bus Element3 : Outport  VectorParamsAs1DForOutWhenUnconnected=off  PortName=OutB  Element=MBrakeL2
  Out Bus Element4 : Outport  VectorParamsAs1DForOutWhenUnconnected=off  PortName=OutB  Element=MBrakeR2
  wires:
  In Bus Element5/1 -> Actuator L1/1(Pedal), Actuator R1/1(Pedal), Actuator R2/1(Pedal), Actuator L2/1(Pedal)
  In Bus Element1/1 -> Terminator/1
  Sensing Torque L1/1(T) -> Out Bus Element2/1
  Sensing Torque R1/1(T) -> Out Bus Element/1
  Sensing Torque L2/1(T) -> Out Bus Element3/1
  Sensing Torque R2/1(T) -> Out Bus Element4/1
  connections:
  Sensing Torque R2/LConn1 -- Disc Brake R2/LConn2
  Sensing Torque R1/LConn1 -- Disc Brake R1/LConn2
  Actuator R1/RConn1 -- Disc Brake R1/LConn1
  Actuator L2/RConn1 -- Disc Brake L2/LConn1
  Actuator L1/RConn1 -- Disc Brake L1/LConn1
  Actuator R2/RConn1 -- Disc Brake R2/LConn1
  R1/RConn1 -- Simscape Bus R1/RConn1
  R2/RConn1 -- Simscape Bus R2/RConn1
  Simscape Bus L2/RConn1 -- L2/RConn1
  Sensing Torque L2/LConn1 -- Disc Brake L2/LConn2
  Simscape Bus L1/RConn1 -- L1/RConn1
  Sensing Torque L1/LConn1 -- Disc Brake L1/LConn2
  Sensing Torque L1/RConn1 -- Simscape Bus L1/LConn1
  Sensing Torque R1/RConn1 -- Simscape Bus R1/LConn1
  Sensing Torque L2/RConn1 -- Simscape Bus L2/LConn1
  Sensing Torque R2/RConn1 -- Simscape Bus R2/LConn1

== system sm_car/Vehicle/Vehicle/Chassis/Aero ==
  note: Lift force acts along the z axis of the frame where the External Force and Torque is attached. Direction is set by the Lift Coefficient.
  note: Drag force acts in the opposite direction of the x-velocity along the x axis of the frame where the External Force and Torque is attached
  fWind : Inport
  External Force Drag and Lift : sm_lib/Forces and Torques/External Force and Torque  EnableForceX=on  EnableForceY=off  EnableForceZ=on  EnableForce=off  ForceResolutionFrame=AttachedFrame  EnableTorqueX=off  EnableTorqueY=off  EnableTorqueZ=off  EnableTorque=off  TorqueResolutionFrame=AttachedFrame
  External Force Wind Gust : sm_lib/Forces and Torques/External Force and Torque  EnableForceX=off  EnableForceY=off  EnableForceZ=off  EnableForce=on  ForceResolutionFrame=World  EnableTorqueX=off  EnableTorqueY=off  EnableTorqueZ=off  EnableTorque=off  TorqueResolutionFrame=AttachedFrame
  Gain : Gain  Gain=0.5 * rho * CL * A
  Gain1 : Gain  Gain=-0.5 * rho * CD * A
  PS-Simulink Converter2 : nesl_utility/PS-Simulink Converter  PhysicalDomain=network_engine_domain  SubClassName=ps_output  LeftPortType=input  RightPortType=output  PseudoPeriodic=off  Frequencies=[]  VectorFormat=1-D array  Unit=1  AffineConversion=off
  Product : Product
  Product1 : Product
  Sign : Signum  ZeroCross=off
  Simulink-PS Converter : nesl_utility/Simulink-PS Converter  PhysicalDomain=network_engine_domain  SubClassName=ps_input  LeftPortType=input  RightPortType=output  PseudoPeriodic=off  Frequencies=[]  NoiseDistribution=none  NoiseParameters=[]  Unit=1  AffineConversion=off  FilteringAndDerivatives=provide  SimscapeFilterOrder=1  InputFilterTimeConstant=0.001  UdotUserProvided=0
  Simulink-PS Converter1 : nesl_utility/Simulink-PS Converter  PhysicalDomain=network_engine_domain  SubClassName=ps_input  LeftPortType=input  RightPortType=output  PseudoPeriodic=off  Frequencies=[]  NoiseDistribution=none  NoiseParameters=[]  Unit=1  AffineConversion=off  FilteringAndDerivatives=provide  SimscapeFilterOrder=1  InputFilterTimeConstant=0.001  UdotUserProvided=0
  Subsystem : Subsystem
  Transform Center of Pressure : sm_lib/Frames and Transforms/Rigid Transform  RotationMethod=None  FollAlignAxisA=+X  BaseAlignAxisA=+Y  FollAlignAxisB=+Y  BaseAlignAxisB=+Z  RotationStandardAxis=+Z  RotationAngle=0.0  RotationAngleUnits=deg  RotationArbitraryAxis=[0 0 1]  RotationSequenceAxes=FollowerAxes  RotationSequence=XYX  RotationSequenceAngles=[0 0 0]  RotationSequenceAnglesUnits=deg  RotationMatrix=[1 0 0; 0 1 0; 0 0 1]  Quaternion=[1 0 0 0]  TranslationMethod=Cartesian  TranslationCartesianOffset=sCentreOfPressure  TranslationCartesianOffsetUnits=m  TranslationStandardAxis=+Z  TranslationStandardOffset=0  TranslationStandardOffsetUnits=m  TranslationROffset=0  TranslationROffsetUnits=m  TranslationThetaOffset=0  TranslationThetaOffsetUnits=deg  TranslationZOffset=0  TranslationZOffsetUnits=m
  Transform Sensor : sm_lib/Frames and Transforms/Transform Sensor  MeasurementFrame=NonRotatingFollower  RotationSequence=XYX  SenseAngle=off  SenseAxis=off  SenseQ=off  SenseR=off  SenseRotationSequence=off  SenseOmegaX=off  SenseOmegaY=off  SenseOmegaZ=off  SenseOmega=off  SenseQDot=off  SenseRDot=off  SenseRotationSequenceDot=off  SenseAlphaX=off  SenseAlphaY=off  SenseAlphaZ=off  SenseAlpha=off  SenseQDDot=off  SenseRDDot=off  SenseX=off  SenseY=off  SenseZ=off  SenseXYZ=off  SenseRad=off  SenseAzim=off  SenseDist=off  SenseInc=off  SenseXDot=on  SenseYDot=off  SenseZDot=off  SenseXYZDot=off  SenseRadDot=off  SenseAzimDot=off  SenseDistDot=off  SenseIncDot=off  SenseXDDot=off  SenseYDDot=off  SenseZDDot=off  SenseXYZDDot=off  SenseRadDDot=off  SenseAzimDDot=off  SenseDistDDot=off  SenseIncDDot=off
  Vis Center of Pressure : sm_lib/Body Elements/Spherical Solid  SphereRadius=rad_hp  SphereRadiusUnits=m  ExportEntireGeometry=off  InertiaType=CalculateFromGeometry  BasedOnType=Density  Density=1000  DensityUnits=kg/m^3  Mass=1  MassUnits=kg  CenterOfMass=[0 0 0]  CenterOfMassUnits=m  MomentsOfInertia=[1 1 1]  MomentsOfInertiaUnits=kg*m^2  ProductsOfInertia=[0 0 0]  ProductsOfInertiaUnits=kg*m^2  GraphicType=FromGeometry  MarkerShape=Sphere  MarkerSize=10  GraphicVisPropType=SimpleVisualProperties  GraphicDiffuseColor=clr_hp  GraphicOpacity=opc_hp  GraphicSpecularColor=[0.5 0.5 0.5 1.0]  GraphicAmbientColor=[0.15 0.15 0.15 1.0]  GraphicEmissiveColor=[0.0 0.0 0.0 1.0]  GraphicShininess=75  DoExposeReferenceFrame=on  SerializedFrames=<Frames/>
  World Frame : sm_lib/Frames and Transforms/World Frame
  A : PMIOPort  Side=Right
  Bus Element Out1 : Outport  VectorParamsAs1DForOutWhenUnconnected=off  PortName=meas  Element=Fx
  Bus Element Out : Outport  VectorParamsAs1DForOutWhenUnconnected=off  PortName=meas  Element=Fz
  wires:
  PS-Simulink Converter2/1 -> Product/1, Product/2, Sign/1
  Product1/1 -> Gain1/1
  Product/1 -> Gain/1, Product1/1
  Sign/1 -> Product1/2
  fWind/1 -> Subsystem/1(RdBus)
  Gain/1 -> Simulink-PS Converter/1, Bus Element Out/1
  Gain1/1 -> Simulink-PS Converter1/1, Bus Element Out1/1
  connections:
  Simulink-PS Converter/RConn1 -- External Force Drag and Lift/LConn2
  Simulink-PS Converter1/RConn1 -- External Force Drag and Lift/LConn1
  Subsystem/RConn1 -- External Force Wind Gust/LConn1
  Transform Center of Pressure/RConn1 -- Vis Center of Pressure/RConn1 -- External Force Wind Gust/RConn1 -- Transform Sensor/RConn1 -- External Force Drag and Lift/RConn1
  Transform Center of Pressure/LConn1 -- A/RConn1
  PS-Simulink Converter2/LConn1 -- Transform Sensor/RConn2
  Transform Sensor/LConn1 -- World Frame/RConn1
